simulink model "lab9_control_optimo"  (R2026b)
settings: Solver=FixedStepDiscrete  StopTime=tiempoFinalLab9  FixedStep=TsLab9
InitFcn:
  | inicializar_simulink_lab9;
values from neighbouring files (symbols this model uses):
  AobservadorLab9 = Aidentificada    [inicializar_simulink_lab9.m]
  AplantaLab9 = Anominal    [inicializar_simulink_lab9.m]
  BobservadorLab9 = Bidentificada    [inicializar_simulink_lab9.m]
  BplantaLab9 = Bnominal    [inicializar_simulink_lab9.m]
  CobservadorLab9 = Cplanta    [inicializar_simulink_lab9.m]
  Cplanta = [0, 1]    [inicializar_simulink_lab9.m]
  Dplanta = 0    [inicializar_simulink_lab9.m]
  finReferenciaLab9 = 0.666    [inicializar_simulink_lab9.m]
  inicioReferenciaLab9 = 0.064    [inicializar_simulink_lab9.m]
  KiLab9 = KoptimaLab9(3)    [inicializar_simulink_lab9.m]
  KxLab9 = KoptimaLab9(1:2)    [inicializar_simulink_lab9.m]
  LobservadorLab9 = place(Aidentificada',      (Cplanta*Aidentificada)', polosObservadorLab9).'    [inicializar_simulink_lab9.m]
  referenciaLab9 = 0.500    (= 0.5)    [inicializar_simulink_lab9.m]
  TsLab9 = 0.002    [inicializar_simulink_lab9.m]
  uMaxLab9 = 1.000    (= 1)    [inicializar_simulink_lab9.m]
  uMinLab9 = -1.000    (= -1)    [inicializar_simulink_lab9.m]
settings Model: Creator=aldop  LastModifiedBy=aldop

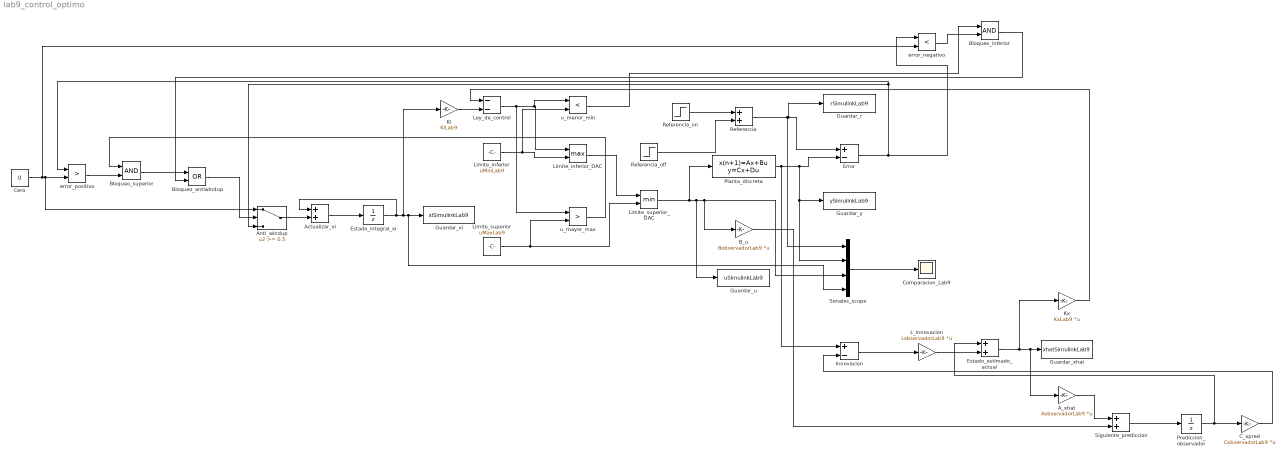
== system lab9_control_optimo ==
  A_xhat : Gain  Gain=AobservadorLab9  Multiplication=Matrix(K*u)
  Actualizar_xi : Sum
  Anti_windup : Switch  Threshold=0.5  SaturateOnIntegerOverflow=off  InputSameDT=off
  B_u : Gain  Gain=BobservadorLab9  Multiplication=Matrix(K*u)
  Bloqueo_antiwindup : Logic  Operator=OR  IconShape=distinctive  AllPortsSameDT=off  OutDataTypeStr=boolean
  Bloqueo_inferior : Logic  IconShape=distinctive  AllPortsSameDT=off  OutDataTypeStr=boolean
  Bloqueo_superior : Logic  IconShape=distinctive  AllPortsSameDT=off  OutDataTypeStr=boolean
  C_xpred : Gain  Gain=CobservadorLab9  Multiplication=Matrix(K*u)
  Cero : Constant  Value=0
  Comparacion_Lab9 : Scope
  Error : Sum  Inputs=+-
  Estado_estimado_actual : Sum
  Estado_integral_xi : UnitDelay  SampleTime=TsLab9
  Guardar_r : ToWorkspace  VariableName=rSimulinkLab9  SaveFormat=Timeseries  SampleTime=-1
  Guardar_u : ToWorkspace  VariableName=uSimulinkLab9  SaveFormat=Timeseries  SampleTime=-1
  Guardar_xhat : ToWorkspace  VariableName=xhatSimulinkLab9  SaveFormat=Timeseries  SampleTime=-1
  Guardar_xi : ToWorkspace  VariableName=xiSimulinkLab9  SaveFormat=Timeseries  SampleTime=-1
  Guardar_y : ToWorkspace  VariableName=ySimulinkLab9  SaveFormat=Timeseries  SampleTime=-1
  Innovacion : Sum  Inputs=+-
  Ki : Gain  Gain=KiLab9
  Kx : Gain  Gain=KxLab9  Multiplication=Matrix(K*u)
  L_innovacion : Gain  Gain=LobservadorLab9  Multiplication=Matrix(K*u)
  Ley_de_control : Sum  Inputs=--
  Limite_inferior : Constant  Value=uMinLab9
  Limite_inferior_DAC : MinMax  Function=max  Inputs=2
  Limite_superior : Constant  Value=uMaxLab9
  Limite_superior_DAC : MinMax  Inputs=2
  Planta_discreta : DiscreteStateSpace  A=AplantaLab9  B=BplantaLab9  C=Cplanta  D=Dplanta  InitialCondition=[0;0]  SampleTime=TsLab9
  Prediccion_observador : UnitDelay  InitialCondition=[0;0]  SampleTime=TsLab9
  Referencia : Sum
  Referencia_off : Step  Time=finReferenciaLab9  FinalValue=-referenciaLab9  SampleTime=TsLab9
  Referencia_on : Step  Time=inicioReferenciaLab9  FinalValue=referenciaLab9  SampleTime=TsLab9
  Senales_scope : Mux
  Siguiente_prediccion : Sum
  error_negativo : RelationalOperator  Operator=<  OutDataTypeStr=boolean  RndMeth=Simplest  InputSameDT=off
  error_positivo : RelationalOperator  Operator=>  OutDataTypeStr=boolean  RndMeth=Simplest  InputSameDT=off
  u_mayor_max : RelationalOperator  Operator=>  OutDataTypeStr=boolean  RndMeth=Simplest  InputSameDT=off
  u_menor_min : RelationalOperator  Operator=<  OutDataTypeStr=boolean  RndMeth=Simplest  InputSameDT=off
  wires:
  Limite_superior_DAC/1 -> Senales_scope/3, B_u/1, Guardar_u/1, Planta_discreta/1
  Limite_inferior_DAC/1 -> Limite_superior_DAC/1
  Referencia_on/1 -> Referencia/1
  Referencia_off/1 -> Referencia/2
  Referencia/1 -> Error/1, Guardar_r/1, Senales_scope/1
  Planta_discreta/1 -> Guardar_y/1, Senales_scope/2, Error/2, Innovacion/1
  Error/1 -> error_positivo/1, Anti_windup/3, error_negativo/1
  Cero/1 -> error_positivo/2, Anti_windup/1, error_negativo/2
  Ley_de_control/1 -> u_menor_min/1, Limite_inferior_DAC/1, u_mayor_max/1
  Limite_superior/1 -> Limite_superior_DAC/2, u_mayor_max/2
  Limite_inferior/1 -> u_menor_min/2, Limite_inferior_DAC/2
  u_mayor_max/1 -> Bloqueo_superior/1
  error_positivo/1 -> Bloqueo_superior/2
  u_menor_min/1 -> Bloqueo_inferior/1
  error_negativo/1 -> Bloqueo_inferior/2
  Bloqueo_superior/1 -> Bloqueo_antiwindup/1
  Bloqueo_inferior/1 -> Bloqueo_antiwindup/2
  Bloqueo_antiwindup/1 -> Anti_windup/2
  Estado_integral_xi/1 -> Senales_scope/4, Guardar_xi/1, Ki/1, Actualizar_xi/1
  Anti_windup/1 -> Actualizar_xi/2
  Actualizar_xi/1 -> Estado_integral_xi/1
  Prediccion_observador/1 -> Estado_estimado_actual/1, C_xpred/1
  C_xpred/1 -> Innovacion/2
  Innovacion/1 -> L_innovacion/1
  L_innovacion/1 -> Estado_estimado_actual/2
  Estado_estimado_actual/1 -> A_xhat/1, Guardar_xhat/1, Kx/1
  Kx/1 -> Ley_de_control/1
  Ki/1 -> Ley_de_control/2
  A_xhat/1 -> Siguiente_prediccion/1
  B_u/1 -> Siguiente_prediccion/2
  Siguiente_prediccion/1 -> Prediccion_observador/1
  Senales_scope/1 -> Comparacion_Lab9/1
